simulink model "Bat"  (R2025b)
settings: Solver=VariableStepAuto  StartTime=0.0  StopTime=inf  FixedStep=ts  RelTol=1e-3  EnableMultiTasking=on
libraries: autolibdcdc x1, autolibdatasheetbattery x1
settings Model: ModifiedByFormat=The MathWorks, Inc.  SimulationMode=accelerator  PauseTimes=10  Creator=The MathWorks, Inc.  LastModifiedBy=The MathWorks, Inc.
settings SolverCC: AlgebraicLoopSolver=TrustRegion  DecoupledContinuousIntegration=on  MaxZcPerStep=1.0
settings DataIOCC: DSMLogging=off  ReturnWorkspaceOutputs=off
settings DebuggingCC: UnconnectedInputMsg=warning  UnconnectedOutputMsg=warning  UnconnectedLineMsg=warning  ArithmeticOperatorsInVariantConditions=warning
settings ModelReferenceCC: EnableRefExpFcnMdlSchedulingChecks=on  PropagateSignalLabelsOutOfModel=off
settings SFSimCC: SimUseLocalCustomCode=off  CustomCodeUndefinedFunction=UseInterfaceOnly
settings RTWCC: RTWUseLocalCustomCode=off  GPUComputeCapability=3.5  DLArmComputeVersion=19.05
settings CodeAppCC: StateflowObjectComments=on
settings GRTTargetCC: TargetLangStandard=C89/C90 (ANSI)
settings ConfigComp: CovMetricSettings=dsw  CovSaveCumulativeToWorkspaceVar=on  CovSaveSingleToWorkspaceVar=on  CovExternalEMLEnable=off
settings SimscapeCC: SimscapeNormalizeSystem=off  SimscapeNominalValues={1, 'bar'; 1, 'cm^3/s'; 1, 'bar*kg/s'; 1, 'kJ/kg'; 1, 'kW'; };

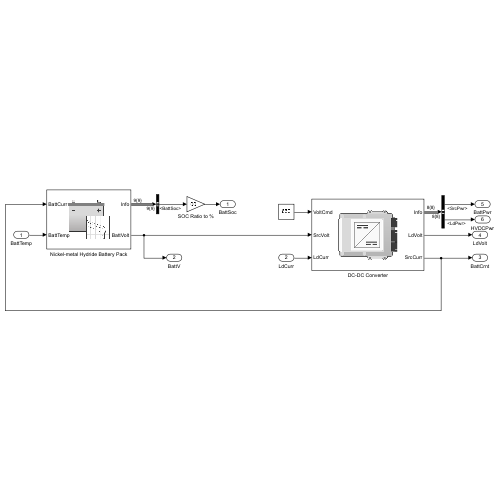
[thumbnail: Simulink's stored preview of the top-level diagram]
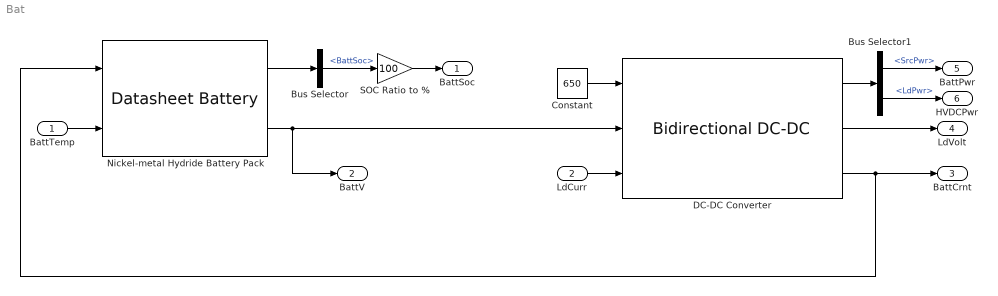
== system Bat ==
  BattTemp : Inport
  LdCurr : Inport  Port=2
  Bus Selector : BusSelector  OutputSignals=BattSoc
  Bus Selector1 : BusSelector  OutputSignals=SrcPwr,LdPwr
  Constant : Constant  Value=650
  DC-DC Converter : autolibdcdc/Bidirectional DC-DC  Tc=1/1000  Vinit=650  Plimit=28e3  param_loss=Single efficiency measurement  eff=98  v_loss_bp=[0 200 400 600 800 1000]  i_loss_bp=[0 25 50 75 100]  losses_table=[100 100 100 100 100;100 150 200 250 300;100 200 300 400 500;100 250 400 550 700;100 300 500 700 900;100 350 600 850 1100]  v_eff_bp=[200 400 600 800 1000]  i_eff_bp=[25 50 75 100]  efficiency_table=[96.2 98.1 98.7 99;98.1 99 99.4 99.5;98.7 99.4 99.6 99.7;99 99.5 99.7 99.8;99.2 99.6 99.7 99.8]  x_v_bp=[-1000 -800 -600 -400 -200 200 400 600 800 1000]  x_i_bp=[-100 -75 -50 -25 25 50 75 100]  x_losses_mat=[200.400801603196 225.67703109328 200.803212851408 201.612903225806 199.999999999997 200 225 200;160.320641282556 180.541624874624 201.005025125625 202.020202020203 200 200 180 160;180.541624874624 180.722891566267 181.086519114686 197.568389057748 194.999999999999 179.999999999997 180 180;201.005025125625 181.086519114686 202.020202020203 193.67991845056 190 200 179.999999999997 200;202.020202020203 197.568389057748 193.67991845056 197.505197505197 190 190 194.999999999999 200;200 194.999999999999 190 190 197.505197505197 193.67991845056 197.568389057748 202.020202020203;200 179.999999999997 200 190 193.67991845056 202.020202020203 181.086519114686 201.005025125625;180 180 179.999999999997 194.999999999999 197.568389057748 181.086519114686 180.722891566267 180.541624874624;160 180 200 200 202.020202020203 201.005025125625 180.541624874624 160.320641282556;200 225 200 199.999999999997 201.612903225806 200.803212851408 225.67703109328 200.400801603196]  RefBlkName='autolibdcdc/Bidirectional DC-DC'  CalLossMapData={'BaseCageProjectFileName','';'BaseMbcProjectFileName','';'TaskName','Calibrate Inverter Loss Map';'ChildTasks',{{'DataName','';'TaskName','Import Loss Data'},{'TaskName','Generate Response Models'},{'TaskName','Generate Calibration'},{'TaskName','Update Block Parameters'}}}
  Nickel-metal Hydride Battery Pack : autolibdatasheetbattery/Datasheet Battery  CapacityCtrl=Parameter  OutputVlt=Filtered  BattChargeMax=6.5  Em=[2.8 3.228 3.284 3.361 3.408 3.427 3.472 3.477 3.493 3.504 3.516 3.528 3.537 3.545 3.555 3.561 3.566 3.576 3.587 3.589 3.594 3.6 3.608 3.61 3.616 3.619 3.626 3.632 3.637 3.64 3.645 3.646 3.652 3.655 3.658 3.661 3.664 3.668 3.673 3.678 3.68 3.681 3.686 3.692 3.699 3.702 3.705 3.71 3.717 3.723 3.728 3.733 3.735 3.742 3.749 3.755 3.761 3.768 3.773 3.78 3.791 3.798 3.798 3.814 3.818 3.825 3.841 3.846 3.855 3.863 3.877 3.885 3.894 3.907 3.919 3.926 3.935 3.944 3.954 3.964 3.974 3.988 3.998 4.014 4.029 4.034 4.047 4.065 4.074 4.086 4.097 4.131 4.126 4.138 4.15 4.18 4.174 4.187 4.207 4.231 4.221]*1.2/4.2  SOCEmBp=[0 0.01 0.02 0.03 0.04 0.05 0.06 0.07 0.08 0.09 0.1 0.11 0.12 0.13 0.14 0.15 0.16 0.17 0.18 0.19 0.2 0.21 0.22 0.23 0.24 0.25 0.26 0.27 0.28 0.29 0.3 0.31 0.32 0.33 0.34 0.35 0.36 0.37 0.38 0.39 0.4 0.41 0.42 0.43 0.44 0.45 0.46 0.47 0.48 0.49 0.5 0.51 0.52 0.53 0.54 0.55 0.56 0.57 0.58 0.59 0.6 0.61 0.62 0.63 0.64 0.65 0.66 0.67 0.68 0.69 0.7 0.71 0.72 0.73 0.74 0.75 0.76 0.77 0.78 0.79 0.8 0.81 0.82 0.83 0.84 0.85 0.86 0.87 0.88 0.89 0.9 0.91 0.92 0.93 0.94 0.95 0.96 0.97 0.98 0.99 1]  RInt="[9.03E-04\t0.00102436\t0.001102155\t0.001157501\t0.001219704\t0.001294037;8.20E-04\t9.46E-04\t0.001004623\t0.001038334\t0.00109789\t0.001176418;7.17E-04\t8.54E-04\t8.82E-04\t8.87E-04\t9.52E-04\t0.001038959;5.80E-04\t7.32E-04\t7.23E-04\t7.03E-04\t7.76E-04\t8.71E-04;4.12E-04\t5.21E-04\t5.13E-04\t5.08E-04\t5.50E-04\t6.38E-04;1.60E-04\t2.05E-04\t1.97E-04\t2.16E-04\t2.10E-04\t2.90E-04;2.94E-04\t3.82E-04\t2.86E-04\t4.39E-04\t4.42E-04\t7.97E-04]"  BattTempBp=[243.1 253.1 263.1 273.1 283.1 298.1 313.1]  SOCRintBp=[0 0.2 0.4 0.6 0.8 1]  Ns=168  Np=1  BattCapInit=6.5*0.6  Tc=1/1000  Vinit=182  RefBlkName='autolibdatasheetbattery/Datasheet Battery'
  SOC Ratio to % : Gain  Gain=100
  BattSoc : Outport  VectorParamsAs1DForOutWhenUnconnected=off
  BattV : Outport  Port=2  VectorParamsAs1DForOutWhenUnconnected=off
  BattCrnt : Outport  Port=3  VectorParamsAs1DForOutWhenUnconnected=off
  LdVolt : Outport  Port=4  VectorParamsAs1DForOutWhenUnconnected=off
  BattPwr : Outport  Port=5  VectorParamsAs1DForOutWhenUnconnected=off
  HVDCPwr : Outport  Port=6  VectorParamsAs1DForOutWhenUnconnected=off
  wires:
  Bus Selector/1 -> SOC Ratio to %/1  "<BattSoc>"
  Nickel-metal Hydride Battery Pack/1 -> Bus Selector/1
  Nickel-metal Hydride Battery Pack/2 -> DC-DC Converter/2, BattV/1
  BattTemp/1 -> Nickel-metal Hydride Battery Pack/2
  DC-DC Converter/3 -> Nickel-metal Hydride Battery Pack/1, BattCrnt/1
  SOC Ratio to %/1 -> BattSoc/1
  Constant/1 -> DC-DC Converter/1
  LdCurr/1 -> DC-DC Converter/3
  DC-DC Converter/1 -> Bus Selector1/1
  DC-DC Converter/2 -> LdVolt/1
  Bus Selector1/1 -> BattPwr/1  "<SrcPwr>"
  Bus Selector1/2 -> HVDCPwr/1  "<LdPwr>"
